simulink library "linear_systems_lib"  (R2018b)
settings: Solver=VariableStepAuto  StartTime=0.0  StopTime=10.0  RelTol=1e-3
settings Model: Creator=Ybeyer  LastModifiedBy=yannic
settings DebuggingCC: LibraryContextMissingDiagnostic=none
settings SFSimCC: SimUseLocalCustomCode=off
settings RTWCC: RTWUseLocalCustomCode=off
settings CodeAppCC: StateflowObjectComments=on

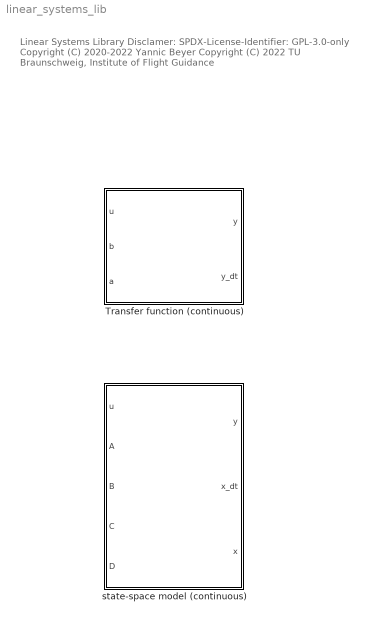
== system linear_systems_lib ==
  note: Linear Systems Library
      |
      | Disclamer:
      | SPDX-License-Identifier: GPL-3.0-only
      |
      | Copyright (C) 2020-2022 Yannic Beyer
      | Copyright (C) 2022 TU Braunschweig, Institute of Flight Guidance
  Transfer function (continuous) : Subsystem
      mask DialogControl DescGroupVar Prompt: Description
      mask DialogControl DescTextVar Prompt: Inputs:
      mask DialogControl Control2 Prompt: u   - input of transfer function
      mask DialogControl Control3 Prompt: b   - coefficients of the numerator transfer function (1st element corresponds to highest exponent)
      mask DialogControl Control4 Prompt: a   - coefficients of the denominator transfer function (1st element corresponds to the highest exponent)
      mask DialogControl Control5 Prompt: Outputs:
      mask DialogControl Control6 Prompt: y   - output of transfer function
      mask DialogControl Control7 Prompt: y_dt   - time-derivative(s) of output of transfer function
  state-space model (continuous) : Subsystem
      mask DialogControl DescGroupVar Prompt: state-space model (continuous)
      mask DialogControl DescTextVar Prompt: can be used with external matrices

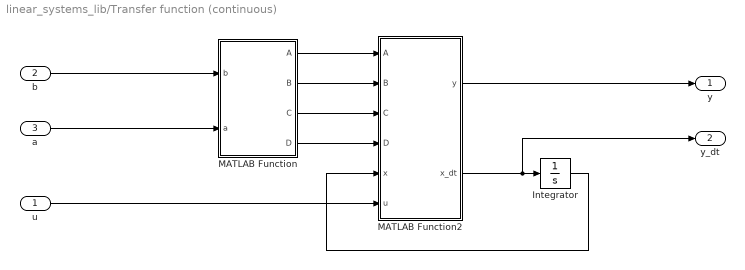
== system linear_systems_lib/Transfer function (continuous) ==
  u : Inport
  b : Inport  Port=2
  a : Inport  Port=3
  Integrator : Integrator
  MATLAB Function : MATLAB Function  TreatAsAtomicUnit=on
  MATLAB Function2 : MATLAB Function  TreatAsAtomicUnit=on
  y : Outport
  y_dt : Outport  Port=2
  wires:
  MATLAB Function/3(C) -> MATLAB Function2/3(C)
  MATLAB Function/2(B) -> MATLAB Function2/2(B)
  MATLAB Function/1(A) -> MATLAB Function2/1(A)
  MATLAB Function2/1(y) -> y/1
  a/1 -> MATLAB Function/2(a)
  Integrator/1 -> MATLAB Function2/5(x)
  MATLAB Function2/2(x_dt) -> y_dt/1, Integrator/1
  b/1 -> MATLAB Function/1(b)
  MATLAB Function/4(D) -> MATLAB Function2/4(D)
  u/1 -> MATLAB Function2/6(u)

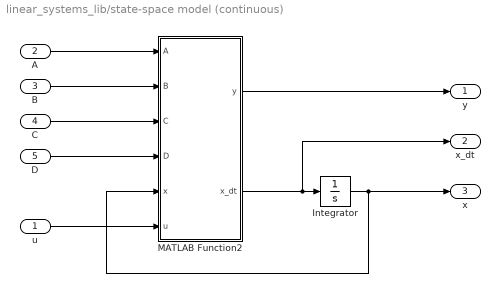
== system linear_systems_lib/state-space model (continuous) ==
  u : Inport
  A : Inport  Port=2
  B : Inport  Port=3
  C : Inport  Port=4
  D : Inport  Port=5
  Integrator : Integrator
  MATLAB Function2 : MATLAB Function  TreatAsAtomicUnit=on
  y : Outport
  x_dt : Outport  Port=2
  x : Outport  Port=3
  wires:
  C/1 -> MATLAB Function2/3(C)
  D/1 -> MATLAB Function2/4(D)
  Integrator/1 -> MATLAB Function2/5(x), x/1
  MATLAB Function2/2(x_dt) -> x_dt/1, Integrator/1
  u/1 -> MATLAB Function2/6(u)
  MATLAB Function2/1(y) -> y/1
  A/1 -> MATLAB Function2/1(A)
  B/1 -> MATLAB Function2/2(B)

== matlab function linear_systems_lib/state-space model (continuous)/MATLAB Function2 ==
  data: A input; B input; C input; D input; x input; u input; y output; x_dt output
function [ y, x_dt ] = fcn( A, B, C, D, x, u ) %#codegen
[ y, x_dt ] = ssOutput( A, B, C, D, x, u );
end

== matlab function linear_systems_lib/Transfer function (continuous)/MATLAB Function ==
  data: b input; A output; a input; B output; C output; D output
function [ A, B, C, D ] = fcn( b, a ) %#codegen
    [ A, B, C, D ] = tf2ssOcf( b, a );
end

== matlab function linear_systems_lib/Transfer function (continuous)/MATLAB Function2 ==
  data: A input; B input; C input; D input; x input; u input; y output; x_dt output
function [ y, x_dt ] = fcn( A, B, C, D, x, u ) %#codegen
[ y, x_dt ] = ssOutput( A, B, C, D, x, u );
end
